simulink model "aula_09"  (R2026a)
settings: Solver=ode45  StopTime=12*tau + 6*theta  MaxStep=tau/20
values from neighbouring files (symbols this model uses):
  gamma = 1/8    (= 0.125)    [Lab11.m]    (also in Lab11_pronto.m; aula08.m; aula08_lab.m; lab09.m)
  Kc = 0.2587    [Lab11.m]    (also in Lab11_pronto.m; aula08.m = 3; aula08_lab.m = 1; lab09.m = M(idx).Kc)
  Kp = 2.721    [Lab11.m]    (also in Lab11_pronto.m; lab09.m)
  tau = -1/alpha    [Lab11.m]    (also in Lab11_pronto.m = 27.21; Lab_7.m; aula08.m = tau_proc; aula08_lab.m = tau_proc)
  Td = 20.66    [Lab11.m]    (also in Lab11_pronto.m; aula08.m = 0; aula08_lab.m = 0; lab09.m = M(idx).Td)
  theta = 2*tau    (= 54.42)    [Lab11.m]    (also in Lab11_pronto.m; lab09.m = 136.05)
  Ti = 53.90    (= 53.9)    [Lab11.m]    (also in Lab11_pronto.m; aula08.m = 1.2; aula08_lab.m = 20; lab09.m = M(idx).Ti)
libraries: slpidlib x1

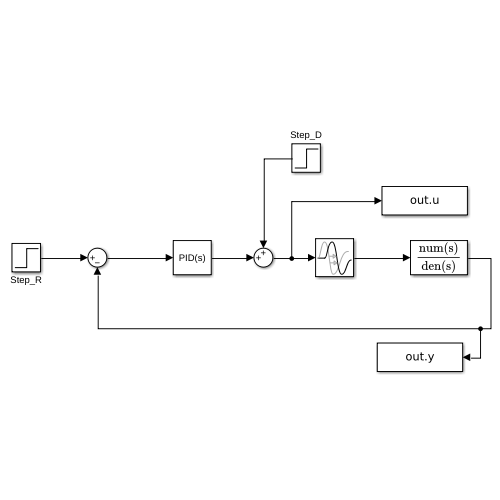
[thumbnail: Simulink's stored preview of the top-level diagram]
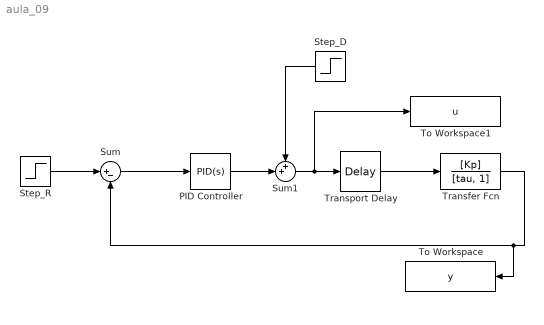
== system aula_09 ==
  PID Controller : slpidlib/PID Controller  Controller=PID  Form=Parallel  TimeDomain=Continuous-time  UseExternalTs=off  SampleTime=-1  IntegratorMethod=Forward Euler  FilterMethod=Forward Euler  ControllerParametersSource=internal  P=Kc  I=Kc/Ti  UseKiTs=off  D=Kc*Td  UseExternalDerivativeSource=off  N=1/(gamma*Td)  UseFilter=on  TunerSelectOption=Transfer Function Based (PID Tuner App)  InitialConditionSource=internal  InitialConditionForIntegrator=0  InitialConditionForFilter=0  DifferentiatorICPrevScaledInput=0  ExternalReset=none  TrackingMode=off  Kt=1  LimitOutput=off  SatLimitsSource=internal  UpperSaturationLimit=inf  LowerSaturationLimit=-inf  LinearizeAsGain=on  AntiWindupMode=none  Kb=1  LimitIntegrator=off  UpperIntegratorSaturationLimit=inf  LowerIntegratorSaturationLimit=-inf  POutMin=[]  POutMax=[]  IOutMin=[]  IOutMax=[]  DOutMin=[]  DOutMax=[]  NOutMin=[]  NOutMax=[]  SumOutMin=[]  SumOutMax=[]  SaturationOutMin=[]  SaturationOutMax=[]  PParamMin=[]  PParamMax=[]  IParamMin=[]  IParamMax=[]  DParamMin=[]  DParamMax=[]  NParamMin=[]  NParamMax=[]  KbParamMin=[]  KbParamMax=[]  KtParamMin=[]  KtParamMax=[]  KbOutMin=[]  KbOutMax=[]  KtOutMin=[]  KtOutMax=[]  IntegratorOutMin=[]  IntegratorOutMax=[]  FilterOutMin=[]  FilterOutMax=[]  SumI1OutMin=[]  SumI1OutMax=[]  SumI2OutMin=[]  SumI2OutMax=[]  SumI3OutMin=[]  SumI3OutMax=[]  SumI4OutMin=[]  SumI4OutMax=[]  SumDOutMin=[]  SumDOutMax=[]  DifferentiatorOutMin=[]  DifferentiatorOutMax=[]  FilterDiffOutCoefMin=[]  FilterDiffOutCoefMax=[]  ReciprocalOutMin=[]  ReciprocalOutMax=[]  SumDenOutMin=[]  SumDenOutMax=[]  SumNumOutMin=[]  SumNumOutMax=[]  DivideOutMin=[]  DivideOutMax=[]  UdiffTsProdOutMin=[]  UdiffTsProdOutMax=[]  NTsProdOutMin=[]  NTsProdOutMax=[]  UintegralTsProdOutMin=[]  UintegralTsProdOutMax=[]  UngainTsProdOutMin=[]  UngainTsProdOutMax=[]  ClampingZeroOutDataTypeStr=Inherit: Inherit via back propagation  ClampingZeroOutMin=[]  ClampingZeroOutMax=[]  FilterDenConstantOutDataTypeStr=Inherit: Inherit via back propagation  FilterDenConstantOutMin=[]  FilterDenConstantOutMax=[]  PCopyOutDataTypeStr=Inherit: Inherit via back propagation  PCopyOutMin=[]  PCopyOutMax=[]  NCopyOutDataTypeStr=Inherit: Inherit via back propagation  NCopyOutMin=[]  NCopyOutMax=[]  IntegratorContinuousStateAttributes=''  IntegratorStateMustResolveToSignalObject=off  IntegratorRTWStateStorageClass=Auto  FilterContinuousStateAttributes=''  FilterStateMustResolveToSignalObject=off  FilterRTWStateStorageClass=Auto  ParallelPVariant=InternalParameters  IdealPVariant=Disabled  IVariant=InternalParameters  DVariant=InternalParameters  IntegratorVariant=Continuous  SatVariant=Disabled  AWVariant=Passthrough  PCopyVariant=Disabled  TRVariant=Disabled  FdbkBlocksVariant=Forward  IdealPFdbkVariant=Disabled  SatFdbkVariant=Disabled  DerivativeFilterVariant=ContFilter  NVariant=InternalParameters  NCopyVariant=Disabled  FilterICVariant=InternalICsFilter  IntegratorICVariant=InternalICs  ExternalResetVariant=Disabled  TRSumVariant=Passthrough  SumFdbkVariant=Disabled  SumVariant=Sum_PID  TsampFilterVariant=InternalTs  TsampNgainVariant=Passthrough  TsampIntegralVariant=Disabled_SignalSpec  ExternalSaturationOutDataTypeStr=Inherit: Same as second input  DerivativeSourceVariant=ErrorSignal  PreIntVariant=InternalPreInt
  Step_D : Step  Time=12*tau  FinalValue=0.05  SampleTime=0
  Step_R : Step  Time=0  FinalValue=0.1  SampleTime=0
  Sum : Sum  Inputs=|+-
  Sum1 : Sum  Inputs=++|
  To Workspace : ToWorkspace  VariableName=y  SampleTime=-1
  To Workspace1 : ToWorkspace  VariableName=u  SampleTime=-1
  Transfer Fcn : TransferFcn  Numerator=[Kp]  Denominator=[tau, 1]
  Transport Delay : TransportDelay  DelayTime=theta
  wires:
  Step_R/1 -> Sum/1
  Sum/1 -> PID Controller/1
  Sum1/1 -> To Workspace1/1, Transport Delay/1
  PID Controller/1 -> Sum1/2
  Step_D/1 -> Sum1/1
  Transport Delay/1 -> Transfer Fcn/1
  Transfer Fcn/1 -> To Workspace/1, Sum/2
